simulink model "testVelocityLin"  (R2019a)
settings: Solver=FixedStepAuto  StartTime=0.0  StopTime=200  FixedStep=DT  RelTol=1e-3
values from neighbouring files (symbols this model uses):
  Cq = saveVarsMat.Cq    [designData.m]
  DT = 0.0080    (= 0.008)    [ObserverWECS_matlab.m]    (also in testExtraTSForVelMdl.m)
  Ng = 97    [ObserverWECS_matlab.m]    (also in param.m = 74.38; parametrs.m; testGradientCq.m)
  omegabar = interp1(LUT_V,LUT_omega,Vbar,'pchip')    [testGradientCq.m]
  R = 33.29    [param.m]    (also in parametrs.m = 63)
  rho = xdotk_1([1,3,4])    [ObserverWECS_matlab.m]    (also in param.m = 1.225; parametrs.m = 1.225; testGradientCq.m = 1.225)
  Rotor_Lambda = [0; 0.1; 0.2; 0.30000000000000004; 0.4; 0.5; 0.60000000000000009;                  0.70000000000000007; 0.8; 0.9; 1; 1.1; 1.2000000000000002;                  1.3; 1.4000000000000001; 1.5; 1.6; 1.7000000000000002;                  1.8; 1.9000000000000001; 2; 2.1; 2.2; 2.3000000000000003;                  2.4000000000000004; 2.5; 2.6; 2.7; 2.8000000000000003;                  2.9000000000000004; 3; ...(+1443 chars)    [designData.m]
  Rotor_Pitch = [-8; -7.8; -7.6; -7.4; -7.2; -7; -6.8; -6.6; -6.4; -6.2;                 -6; -5.8; -5.6; -5.4; -5.1999999999999993; -5; -4.8; -4.6;                 -4.4; -4.1999999999999993; -4; -3.8; -3.5999999999999996;                 -3.3999999999999995; -3.1999999999999993; -3; -2.8; -2.5999999999999996;                 -2.3999999999999995; -2.1999999999999993; -2; -1.7999999999999998;                 -1.599 ...(+1852 chars)    [designData.m]
  tau_g = 0.02    [param.m]    (also in parametrs.m = 0.01; testGradientCq.m = 0.01)
undefined symbols (not defined in the file or in its folder): Drivetrain, Lin_points
settings Model: ExtModeTrigMode=oneshot  ExtModeArmWhenConnect=off  Creator=Hazim Namik  LastModifiedBy=ditt_aj
settings DataIOCC: LimitDataPoints=on  SaveFormat=Array  ReturnWorkspaceOutputs=off
settings OptimizationCC: BlockReduction=off  BooleanDataType=off  LifeSpan=inf
settings DebuggingCC: SaveWithParameterizedLinksMsg=none  UnderspecifiedInitializationDetection=Classic  MergeDetectMultiDrivingBlocksExec=none  SignalResolutionControl=TryResolveAllWithWarning  SFUnexpectedBacktrackingDiag=warning  SFNoUnconditionalDefaultTransitionDiag=warning  SFExecutionAtInitializationDiag=none  ArithmeticOperatorsInVariantConditions=warning
settings HardwareCC: ProdBitPerPointer=32  ProdBitPerSizeT=32  ProdBitPerPtrDiffT=32  ProdLargestAtomicFloat=None  ProdIntDivRoundTo=Undefined  ProdEndianess=Unspecified  ProdWordSize=32  ProdHWDeviceType=32-bit Generic  TargetUnknown=on
settings ModelReferenceCC: PropagateSignalLabelsOutOfModel=off
settings SFSimCC: SimUseLocalCustomCode=off
settings RTWCC: RTWUseLocalCustomCode=off
settings CodeAppCC: StateflowObjectComments=on
settings GRTTargetCC: TargetLangStandard=C89/C90 (ANSI)  GeneratePreprocessorConditionals=Disable all
settings ConfigComp: CovMetricSettings=dw  CovHtmlReporting=on  CovSaveCumulativeToWorkspaceVar=on  CovSaveSingleToWorkspaceVar=on  CovExternalEMLEnable=off

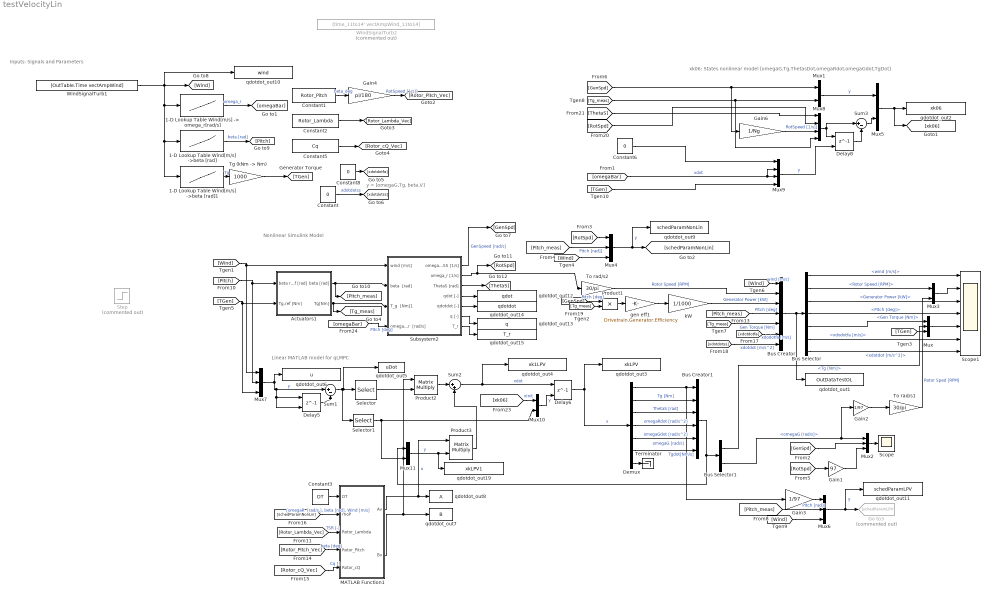
== system testVelocityLin ==
  note: xk06: States nonlinear model [omegaG,Tg,ThetasDot,omegaRdot,omegaGdot,TgDot]
  note: Linear MATLAB model for qLMPC
  note: Inputs: Signals and Parameters
  note: Nonlinear Simulink Model
  note: y = [omegaG,Tg, beta,V]
  "1-D Lookup Table Wind[m/s] -> omega_r[rad/s]" : Lookup_n-D  NumberOfTableDimensions=1  BreakpointsForDimension1=Lin_points.V  BreakpointsForDimension2=Rotor_Lambda  Table=Lin_points.RSpeed  InternalRulePriority=Speed  RndMeth=Simplest  InputSameDT=on
  1-D Lookup Table Wind[m/s] ->beta [rad] : Lookup_n-D  NumberOfTableDimensions=1  BreakpointsForDimension1=Lin_points.V  BreakpointsForDimension2=Rotor_Lambda  Table=Lin_points.Pitch  InternalRulePriority=Speed  RndMeth=Simplest  InputSameDT=on
  1-D Lookup Table Wind[m/s] ->beta [rad]1 : Lookup_n-D  NumberOfTableDimensions=1  BreakpointsForDimension1=Lin_points.V  BreakpointsForDimension2=Rotor_Lambda  Table=Lin_points.Torque  InternalRulePriority=Speed  RndMeth=Simplest  InputSameDT=on
  Actuators1 : Subsystem
  Bus Creator : BusCreator  Inputs=7
  Bus Creator1 : BusCreator  Inputs=6
  Bus Selector : BusSelector  OutputSignals=wind [m/s],Rotor Speed [RPM],Generator Power [kW],Pitch [deg],Gen Torque [Nm],xdodotfa [m/s],xdotdot [m/s^2]
  Bus Selector1 : BusSelector  OutputSignals=Tg [Nm],omegaG [rad/s]
  Constant : Constant  Value=0
  Constant1 : Constant  Value=Rotor_Pitch
  Constant2 : Constant  Value=Rotor_Lambda
  Constant3 : Constant  Value=DT
  Constant5 : Constant  Value=Cq
  Constant6 : Constant  Value=0
  Constant8 : Constant  Value=0
  Delay5 : Delay  DelayLength=1  InitialConditionSource=Input port  InitialCondition=[0, Lin_points.Torque(1)]
      settings: InputPortMap=u0,p4
  Delay6 : Delay  DelayLength=1  InitialConditionSource=Input port
      settings: InputPortMap=u0,p4
  Delay8 : Delay  DelayLength=1  InitialConditionSource=Input port  InitialCondition=[0,omegabar]
      settings: InputPortMap=u0,p4
  Demux : Demux  Outputs=7
  Gain1 : Gain  Gain=97
  Gain2 : Gain  Gain=1/97
  Gain3 : Gain  Gain=1/97
  Gain4 : Gain  Gain=pi/180
  Gain6 : Gain  Gain=1/Ng
  Go to3 : Goto  Commented=on  GotoTag=schedParamLPV
  MATLAB Function1 : MATLAB Function  TreatAsAtomicUnit=on
  Mux{,2,4,6..7} (5 alike) : Mux  Inputs=3
  Mux{1,3,5,10..11} (5 alike) : Mux  Inputs=2
  Mux8 : Mux
  Mux9 : Mux
  Product1 : Product  RndMeth=Zero
  Product2 : Product  Multiplication=Matrix(*)  RndMeth=Zero
  Product3 : Product  Multiplication=Matrix(*)  RndMeth=Zero
  Scope : Scope
  Scope1 : Scope  NumInputPorts=7
      settings: Tag=Scope
  Selector : Selector  InputPortWidth=3  IndexOptions=Index vector (dialog)  Indices=[2 3]  OutputSizes=1
  Selector1 : Selector  InputPortWidth=3  IndexOptions=Index vector (dialog)  Indices=1  OutputSizes=1
  Step : Step  Commented=on  Time=5*DT  Before=12  After=13  SampleTime=0
  Subsystem2 : Subsystem
  Sum1 : Sum  Inputs=|+-
  Sum2 : Sum  Inputs=|++
  Sum3 : Sum  Inputs=|+-
  Terminator : Terminator
  "Tg (kNm -> Nm)" : Gain  Gain=1000
  To rad/s1 : Gain  Gain=30/pi
  To rad/s2 : Gain  Gain=30/pi
  WindSignalTurb1 : FromWorkspace  VariableName=[OutTable.Time vectAmpWind]  SampleTime=DT  OutputAfterFinalValue=Holding final value
  WindSignalTurb2 : FromWorkspace  Commented=on  VariableName=[time_11to14' vectAmpWind_11to14]  SampleTime=DT  OutputAfterFinalValue=Holding final value
  gen eff1 : Gain  Gain=Drivetrain.Generator.Efficiency
  kW : Gain  Gain=1/1000
  qdotdot_out1 : ToWorkspace  VariableName=OutDataTestOL  SampleTime=-1
  qdotdot_out10 : ToWorkspace  VariableName=wind  SampleTime=-1
  qdotdot_out11 : ToWorkspace  VariableName=schedParamLPV  SampleTime=-1
  qdotdot_out12 : ToWorkspace  VariableName=qdot  SampleTime=-1
  qdotdot_out13 : ToWorkspace  VariableName=q  SampleTime=-1
  qdotdot_out14 : ToWorkspace  VariableName=qdotdot  SampleTime=-1
  qdotdot_out15 : ToWorkspace  VariableName=T_r  SampleTime=-1
  qdotdot_out19 : ToWorkspace  VariableName=xkLPV1  SampleTime=-1
  qdotdot_out2 : ToWorkspace  VariableName=xk06  SampleTime=-1
  qdotdot_out3 : ToWorkspace  VariableName=xkLPV  SampleTime=-1
  qdotdot_out4 : ToWorkspace  VariableName=xk1LPV  SampleTime=-1
  qdotdot_out5 : ToWorkspace  VariableName=uDot  SampleTime=-1
  qdotdot_out6 : ToWorkspace  VariableName=u  SampleTime=-1
  qdotdot_out7 : ToWorkspace  VariableName=B  SampleTime=-1
  qdotdot_out8 : ToWorkspace  VariableName=A  SampleTime=-1
  qdotdot_out9 : ToWorkspace  VariableName=schedParamNonLin  SampleTime=-1
  wires:
  1-D Lookup Table Wind[m/s] ->beta [rad]1/1 -> "Tg (kNm -> Nm)"/1  "Tg"
  "1-D Lookup Table Wind[m/s] -> omega_r[rad/s]"/1 -> [omegaBar]  "omega_r"
  1-D Lookup Table Wind[m/s] ->beta [rad]/1 -> [Pitch]  "beta [rad]"
  Constant2/1 -> [Rotor_Lambda_Vec]
  Constant1/1 -> Gain4/1  "beta_deg"
  Constant5/1 -> [Rotor_cQ_Vec]
  WindSignalTurb1/1 -> qdotdot_out10/1, 1-D Lookup Table Wind[m/s] ->beta [rad]1/1, 1-D Lookup Table Wind[m/s] ->beta [rad]/1, "1-D Lookup Table Wind[m/s] -> omega_r[rad/s]"/1, [Wind]
  "Tg (kNm -> Nm)"/1 -> [TGen]
  Bus Selector/6 -> Scope1/6  "<xdodotfa [m/s]>"
  Actuators1/1(beta [rad]) -> [Pitch_meas], Subsystem2/2(beta  [rad])
  To rad/s2/1 -> Bus Creator/2  "Rotor Speed [RPM]"
  [Tg_meas] -> Bus Creator/5  "Gen Torque [Nm]"
  [Wind] -> Subsystem2/1(wind [m/s]), Mux7/1
  Product1/1 -> gen eff1/1
  [xdotdotfa] -> Bus Creator/6  "xdodotfa [m/s]"
  [Pitch_meas] -> Bus Creator/4  "Pitch [deg]"
  Subsystem2/2(omega_r [1/s]) -> [RotSpd], To rad/s2/1
  [xdotdotss] -> Bus Creator/7  "xdotdot [m/s^2]"
  Constant/1 -> [xdotdotss]  "xdotdotss"
  Subsystem2/1(omega_g HSS [1/s]) -> [GenSpd]  "GenSpeed [rad/s]"
  [Wind] -> Bus Creator/1  "wind [m/s]"
  kW/1 -> Bus Creator/3  "Generator Power [kW]"
  Actuators1/2(Tg[Nm]) -> Subsystem2/3(T_g  [Nm]1), [Tg_meas]
  Bus Creator/1 -> Bus Selector/1, qdotdot_out1/1
  Constant8/1 -> [xdotdotfa]
  gen eff1/1 -> kW/1
  Subsystem2/3(ThetaS [rad]) -> [ThetaS]
  Bus Selector/7 -> Scope1/7  "<xdotdot [m/s^2]>"
  Bus Selector/4 -> Scope1/4  "<Pitch [deg]>"
  Bus Selector/3 -> Scope1/3  "<Generator Power [kW]>"
  Bus Selector/1 -> Scope1/1  "<wind [m/s]>"
  Sum3/1 -> Mux5/2
  Mux5/1 -> [xk06], qdotdot_out2/1
  Delay8/1 -> Sum3/2
  [Tg_meas] -> Mux1/2, Mux8/4
  [RotSpd] -> Mux8/2
  [ThetaS] -> Mux8/1
  Mux8/1 -> Sum3/1, Delay8/1
  [GenSpd] -> Gain6/1, Mux1/1
  Mux1/1 -> Mux5/1  "y"
  [RotSpd] -> Mux4/1
  [Pitch_meas] -> Mux4/2  "Pitch [rad]]"
  [Wind] -> Mux4/3
  Mux4/1 -> qdotdot_out9/1, [schedParamNonLin]  "y"
  [Pitch] -> Mux7/2, Actuators1/1(beta ref [rad])
  [TGen] -> Mux7/3, Actuators1/2(Tg,ref [Nm])
  Constant3/1 -> MATLAB Function1/1(DT)
  [Rotor_cQ_Vec] -> MATLAB Function1/5(Rotor_cQ)  "Cq []"
  [Rotor_Pitch_Vec] -> MATLAB Function1/4(Rotor_Pitch)  "beta [deg]"
  [Rotor_Lambda_Vec] -> MATLAB Function1/3(Rotor_Lambda)  "TSR [-]"
  [schedParamNonLin] -> MATLAB Function1/2(rhoP)  "[omegaR  [rad/s,], beta [rad], Wind [m/s]"
  MATLAB Function1/1(Av) -> Product3/1, qdotdot_out8/1  "u"
  Mux7/1 -> Delay5/1, Delay5/2, Sum1/1, qdotdot_out6/1  "y"
  Delay5/1 -> Sum1/2
  Product2/1 -> Sum2/1
  Sum2/1 -> Delay6/1, qdotdot_out4/1  "xdot"
  Delay6/1 -> Demux/1, qdotdot_out3/1  "x"
  Product3/1 -> Sum2/2
  Gain6/1 -> Mux8/3  "RotSpeed [1/s]]"
  Mux9/1 -> Delay8/2  "y"
  [omegaBar] -> Subsystem2/4(omega_r  [rad/s])  "Pitch [deg]"
  [GenSpd] -> Product1/1  "Pitch [deg]"
  [Tg_meas] -> Product1/2
  Demux/1 -> Gain3/1, Bus Creator1/1  "omegaG [rad/s]"
  Demux/2 -> Bus Creator1/2  "Tg [Nm]"
  Demux/3 -> Bus Creator1/3  "ThetaS [rad]"
  Demux/4 -> Bus Creator1/4  "omegaRdot [rad/s^2]"
  Demux/5 -> Bus Creator1/5  "omegaGdot [rad/s^2]"
  Demux/6 -> Bus Creator1/6  "Tgdot[Nm/s]"
  Bus Creator1/1 -> Mux11/1, Bus Selector1/1
  Bus Selector1/1 -> Mux/2  "<Tg [Nm]>"
  Mux/1 -> Scope1/5
  Bus Selector/5 -> Mux/1  "<Gen Torque [Nm]>"
  Sum1/1 -> Selector1/1, Selector/1, qdotdot_out5/1
  [TGen] -> Mux/3
  Bus Selector1/2 -> Gain2/1, Mux2/1  "<omegaG [rad/s]>"
  [GenSpd] -> Mux2/2
  [RotSpd] -> Gain1/1
  Gain1/1 -> Mux2/3
  Mux2/1 -> Scope/1
  Mux3/1 -> Scope1/2
  Bus Selector/2 -> Mux3/1  "<Rotor Speed [RPM]>"
  Gain2/1 -> To rad/s1/1
  To rad/s1/1 -> Mux3/2  "Rotor Sped [RPM]"
  [Wind] -> Mux6/3
  Mux6/1 -> qdotdot_out11/1, Go to3/1  "y"
  Gain3/1 -> Mux6/1
  [Pitch_meas] -> Mux6/2  "Pitch [rad]]"
  Subsystem2/4(qdot [-]) -> qdotdot_out12/1
  Subsystem2/6(q [-]) -> qdotdot_out13/1
  Subsystem2/5(qdotdot [-]) -> qdotdot_out14/1
  [omegaBar] -> Mux9/2, Mux9/3  "xdot"
  [TGen] -> Mux9/4
  Constant6/1 -> Mux9/1
  Subsystem2/7(T_r) -> qdotdot_out15/1
  [xk06] -> Mux10/1  "xInit"
  Mux10/1 -> Delay6/2  "y"
  Selector1/1 -> Mux11/2, Mux10/2
  MATLAB Function1/2(Bv) -> Product2/1, qdotdot_out7/1
  Selector/1 -> Product2/2
  Mux11/1 -> qdotdot_out19/1, Product3/2  "y"
  Demux/7 -> Terminator/1
  Gain4/1 -> [Rotor_Pitch_Vec]  "RotSpeed [1/s]]"

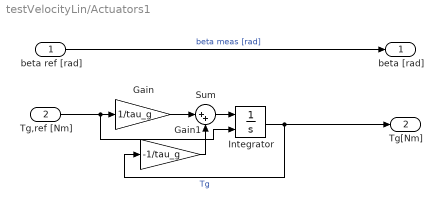
== system testVelocityLin/Actuators1 ==
  beta ref [rad] : Inport
  Tg,ref [Nm] : Inport  Port=2
  Gain : Gain  Gain=1/tau_g
  Gain1 : Gain  Gain=-1/tau_g
  Integrator : Integrator  InitialConditionSource=external
  Sum : Sum  Inputs=|++
  beta [rad] : Outport
  Tg[Nm] : Outport  Port=2
  wires:
  Tg,ref [Nm]/1 -> Integrator/2, Gain/1
  Integrator/1 -> Gain1/1, Tg[Nm]/1  "Tg"
  beta ref [rad]/1 -> beta [rad]/1  "beta meas [rad]"
  Gain/1 -> Sum/1
  Sum/1 -> Integrator/1
  Gain1/1 -> Sum/2

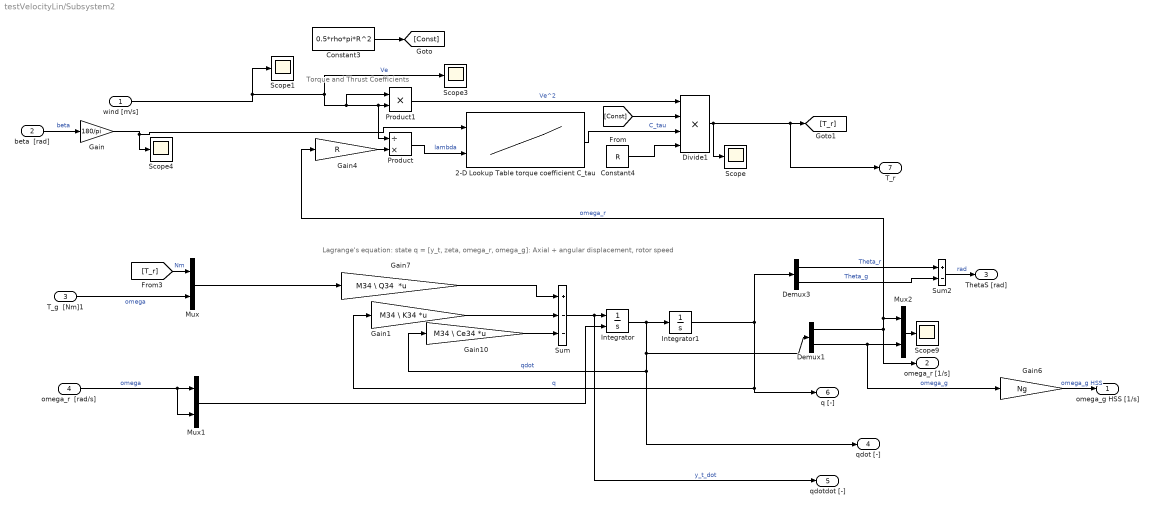
== system testVelocityLin/Subsystem2 ==
  note: Torque and Thrust Coefficients
  note: Lagrange's equation: state q = [y_t, zeta, omega_r, omega_g]: Axial + angular displacement, rotor speed
  wind [m/s] : Inport
  beta  [rad] : Inport  Port=2
  T_g  [Nm]1 : Inport  Port=3
  omega_r  [rad/s] : Inport  Port=4
  2-D Lookup Table torque coefficient C_tau : Lookup_n-D  BreakpointsForDimension1=Rotor_Pitch  BreakpointsForDimension2=Rotor_Lambda  Table=Cq  InterpMethod=Cubic spline  ExtrapMethod=Cubic spline  InternalRulePriority=Speed  RndMeth=Simplest  InputSameDT=on
  Constant3 : Constant  Value=0.5*rho*pi*R^2
  Constant4 : Constant  Value=R
  Demux1 : Demux  Outputs=2
  Demux3 : Demux  Outputs=2
  Divide1 : Product  Inputs=****
  Gain : Gain  Gain=180/pi
  Gain1 : Gain  Gain=M34 \ K34  Multiplication=Matrix(K*u)
  Gain10 : Gain  Gain=M34 \ Ce34  Multiplication=Matrix(K*u)
  Gain4 : Gain  Gain=R
  Gain6 : Gain  Gain=Ng
  Gain7 : Gain  Gain=M34 \ Q34  Multiplication=Matrix(K*u)
  Integrator : Integrator  InitialConditionSource=external  InitialCondition=[0.5, 0.5]
  Integrator1 : Integrator  InitialCondition=[0,0]
  Mux : Mux  Inputs=2
  Mux1 : Mux  Inputs=2
  Mux2 : Mux  Inputs=2
  Product : Product  Inputs=/*
  Product1 : Product  Inputs=**
  Scope{,1,3..4,9} (5 alike) : Scope
  Sum : Sum  Inputs=+--
  Sum2 : Sum  Inputs=+-
  omega_g HSS [1/s] : Outport
  omega_r [1/s] : Outport  Port=2
  ThetaS [rad] : Outport  Port=3
  qdot [-] : Outport  Port=4
  qdotdot [-] : Outport  Port=5
  q [-] : Outport  Port=6
  T_r : Outport  Port=7
  wires:
  Constant4/1 -> Divide1/4
  wind [m/s]/1 -> Product1/1, Product1/2, Product/1, Scope3/1, Scope1/1  "Ve"
  Gain4/1 -> Product/2
  Divide1/1 -> Scope/1, T_r/1, [T_r]
  [Const] -> Divide1/2
  2-D Lookup Table torque coefficient C_tau/1 -> Divide1/3  "C_tau"
  Gain1/1 -> Sum/2
  Gain7/1 -> Sum/1
  Mux/1 -> Gain7/1
  Integrator1/1 -> Demux3/1, q [-]/1, Gain1/1  "q"
  Demux1/1 -> omega_r [1/s]/1, Gain4/1, Mux2/1  "omega_r"
  Demux1/2 -> Gain6/1, Mux2/2  "omega_g"
  beta  [rad]/1 -> Gain/1  "beta"
  Product/1 -> 2-D Lookup Table torque coefficient C_tau/2  "lambda"
  Product1/1 -> Divide1/1  "Ve^2"
  Integrator/1 -> Integrator1/1, Demux1/1, qdot [-]/1, Gain10/1  "qdot"
  Demux3/1 -> Sum2/1  "Theta_r"
  Demux3/2 -> Sum2/2  "Theta_g"
  Gain10/1 -> Sum/3
  Gain6/1 -> omega_g HSS [1/s]/1  "omega_g HSS"
  Constant3/1 -> [Const]
  Mux2/1 -> Scope9/1
  Sum/1 -> qdotdot [-]/1, Integrator/1  "y_t_dot"
  Sum2/1 -> ThetaS [rad]/1  "rad"
  Gain/1 -> 2-D Lookup Table torque coefficient C_tau/1, Scope4/1
  omega_r  [rad/s]/1 -> Mux1/2, Mux1/1  "omega"
  Mux1/1 -> Integrator/2
  [T_r] -> Mux/1  "Nm"
  T_g  [Nm]1/1 -> Mux/2  "omega"

== matlab function testVelocityLin/MATLAB Function1 ==
  settings: updateMethod=DISCRETE
  data: DT input; rhoP input; Av output; Rotor_Lambda input; Rotor_Pitch input; Rotor_cQ input; Bv output
function [Av,Bv] = ABqLd_WT(DT,rhoP,Rotor_Lambda,Rotor_Pitch,Rotor_cQ)
% ABqLd calculates system (A) and input (B) matrix for quasiLPV
% representation from ABgL and augments the states with integrating
% disturbances.
%
% Inputs: * DT: Sampling time
%         * rho: Scheduling parameter vector: rho = V
%
% Outputs: * A: Augmented system matrix A(rho) at current rho
%          * B: Augmented Input matrix B(rho) at current rho

% Pablo S.G. Cisneros, Herbert Werner, ICS TUHH

[Arho,Brho] = ABqL_WT(rhoP,Rotor_Lambda,Rotor_Pitch,Rotor_cQ);
%[Arho,Brho] = ABqL_WT_beta(rhoP,Rotor_Lambda,Rotor_Pitch,Rotor_cQ);
%[Arho, Brho, ~, ~, dTrdomega, Tr, dTrdV] = ABqL_WT_KMC(rhoP,Rotor_Lambda,Rotor_Pitch,Rotor_cQ);

%% Calculate discrete forms of A,B
A2 = Arho*Arho;
A3 = Arho*A2;
Apre = (1.0/24.0)*DT^4*A3+(1.0/6.0)*DT^3*A2+0.5*DT^2*Arho+DT*eye(size(Arho));

%% Finish calculation of A,B
Ak = Apre*Arho + eye(size(Arho));
Bk = Apre*Brho;

%% Calculate new matrices augmented system
ny = 2; %
nx = size(Arho,1);
nyvec = nx-1:nx; % 
nd = 1;% B: columns disturbance input
nuvec = 2:3; % B: columns control input
Cdiag = diag([97,1]); %eye(ny); %diag([97,1]);

A = [eye(2) Cdiag* Ak(3:4,:);
    zeros(size(Ak,1),ny), Ak];

B = [Cdiag* Bk(3:4,2:3); Bk(:,2:3)];
Bv1 = [Cdiag* Bk(3:4,1); Bk(:,1)];

Av = [A,Bv1; [zeros(nd,(nx+ny)) 0 *eye(nd)]];
Bv = [B; zeros(nd, size(B,2))];


end
